simulink model "sys1"  (R2023b)
settings: Solver=VariableStepAuto  StartTime=0.0  StopTime=30e-3  RelTol=1e-3
InitFcn:
  | fs = 100e6;
  | ts = 1 / fs;
values from neighbouring files (symbols this model uses):
  c = 3e8    (= 300000000)    [init_param.m]
  H_az1 = zeros(numSamples,numPulses)    [init_param.m]
  H_az2 = zeros(numSamples,numPulses)    [init_param.m]
  H_ref = fft(conj(fliplr(txChirp)), numSamples)    [init_param.m]
  rawData = rawData + 0.01 * (randn(size(rawData)) + 1j * randn(size(rawData)))    [init_param.m]
  x1 = zeros(size(rawData))    [main.m]
  x2 = zeros(size(x1))    [main.m]
  x3 = zeros(size(x2))    [main.m]
  x4 = zeros(size(x3))    [main.m]
  x5 = zeros(size(x4))    [main.m]
  x6 = zeros(size(x5))    [main.m]
  xx4 = zeros(size(xx3))    [main.m]
  xx5 = zeros(size(xx4))    [main.m]
  xx6 = zeros(size(xx5))    [main.m]
undefined symbols (not defined in the file or in its folder): ffva1156, w2, w3, w4, w5, w6, w7, w8, w9, ww2, ww3, ww4, ww5, ww6, ww7, ww8, ww9, xcku095
libraries: hdlBasic x917, hdlDSPIP x18, dspsrcs4 x12, vmcUtilities x1
(part 9 of 9)

== system sys1/SAR/stream/stream_ifft/stage1/delay/delay1 ==
  in : Inport
  Constant1 : hdlBasic/Constant  const=1  gui_display_data_type=Boolean  arith_type=Boolean  n_bits=16  bin_pt=14  preci_type=Single  exp_width=8  frac_width=24  explicit_period=on  period=ts  XmcBlockStatus=1  maskContainerNames=tabcontainer1  block_type=constant  block_config=sysgen:Constant_config
  Constant3 : hdlBasic/Constant  const=1  gui_display_data_type=Boolean  arith_type=Boolean  n_bits=16  bin_pt=14  preci_type=Single  exp_width=8  frac_width=24  explicit_period=on  period=ts  XmcBlockStatus=1  maskContainerNames=tabcontainer1  block_type=constant  block_config=sysgen:Constant_config
  FIFO : hdlBasic/FIFO  mem_type=Block RAM  performance_options=Standard_FIFO  embedded_registers=off  depth=1K  use_asym_data_widths=off  asym_read_width=32  percent_nbits=1  rst=off  rst_latency=3  en=off  use_dcount=off  use_percent_full_port=off  use_almost_empty=off  almost_empty_thresh=2  use_almost_full=on  use_rd_rst_busy=off  use_wr_rst_busy=off  almost_full_thresh=2^10-3  almost_empty_offset=[]  almost_full_offset=[]  explicit_period=off  period=[]  store_only_valid=[]  init_zero=[]  simulation_type=fast_sim  XmcBlockStatus=1  maskContainerNames=tabcontainer1  block_type=fifo  block_config=sysgen:FIFO_config  block_width=538  block_height=997
      settings: infoedit=[]
  Register2 : hdlBasic/Register  init=0  rst=off  en=on  XmcBlockStatus=1  maskContainerNames=tabcontainer1  block_type=register  block_config=sysgen:Register_config
  out : Outport
  wires:
  FIFO/4 -> Register2/2
  Constant1/1 -> Register2/1
  Register2/1 -> FIFO/3
  Constant3/1 -> FIFO/2
  in/1 -> FIFO/1
  FIFO/1 -> out/1

== system sys1/SAR/stream/stream_ifft/stage2/delay/delay ==
  in : Inport
  Constant1 : hdlBasic/Constant  const=1  gui_display_data_type=Boolean  arith_type=Boolean  n_bits=16  bin_pt=14  preci_type=Single  exp_width=8  frac_width=24  explicit_period=on  period=ts  XmcBlockStatus=1  maskContainerNames=tabcontainer1  block_type=constant  block_config=sysgen:Constant_config
  Constant3 : hdlBasic/Constant  const=1  gui_display_data_type=Boolean  arith_type=Boolean  n_bits=16  bin_pt=14  preci_type=Single  exp_width=8  frac_width=24  explicit_period=on  period=ts  XmcBlockStatus=1  maskContainerNames=tabcontainer1  block_type=constant  block_config=sysgen:Constant_config
  FIFO : hdlBasic/FIFO  mem_type=Block RAM  performance_options=Standard_FIFO  embedded_registers=off  depth=2K  use_asym_data_widths=off  asym_read_width=32  percent_nbits=1  rst=off  rst_latency=3  en=off  use_dcount=off  use_percent_full_port=off  use_almost_empty=off  almost_empty_thresh=2  use_almost_full=on  use_rd_rst_busy=off  use_wr_rst_busy=off  almost_full_thresh=2^11-3  almost_empty_offset=[]  almost_full_offset=[]  explicit_period=off  period=[]  store_only_valid=[]  init_zero=[]  simulation_type=fast_sim  XmcBlockStatus=1  maskContainerNames=tabcontainer1  block_type=fifo  block_config=sysgen:FIFO_config  block_width=538  block_height=997
      settings: infoedit=[]
  Register2 : hdlBasic/Register  init=0  rst=off  en=on  XmcBlockStatus=1  maskContainerNames=tabcontainer1  block_type=register  block_config=sysgen:Register_config
  out : Outport
  wires:
  FIFO/4 -> Register2/2
  Constant1/1 -> Register2/1
  Register2/1 -> FIFO/3
  Constant3/1 -> FIFO/2
  in/1 -> FIFO/1
  FIFO/1 -> out/1

== system sys1/SAR/stream/stream_ifft/stage2/delay/delay1 ==
  in : Inport
  Constant1 : hdlBasic/Constant  const=1  gui_display_data_type=Boolean  arith_type=Boolean  n_bits=16  bin_pt=14  preci_type=Single  exp_width=8  frac_width=24  explicit_period=on  period=ts  XmcBlockStatus=1  maskContainerNames=tabcontainer1  block_type=constant  block_config=sysgen:Constant_config
  Constant3 : hdlBasic/Constant  const=1  gui_display_data_type=Boolean  arith_type=Boolean  n_bits=16  bin_pt=14  preci_type=Single  exp_width=8  frac_width=24  explicit_period=on  period=ts  XmcBlockStatus=1  maskContainerNames=tabcontainer1  block_type=constant  block_config=sysgen:Constant_config
  FIFO : hdlBasic/FIFO  mem_type=Block RAM  performance_options=Standard_FIFO  embedded_registers=off  depth=2K  use_asym_data_widths=off  asym_read_width=32  percent_nbits=1  rst=off  rst_latency=3  en=off  use_dcount=off  use_percent_full_port=off  use_almost_empty=off  almost_empty_thresh=2  use_almost_full=on  use_rd_rst_busy=off  use_wr_rst_busy=off  almost_full_thresh=2^11-3  almost_empty_offset=[]  almost_full_offset=[]  explicit_period=off  period=[]  store_only_valid=[]  init_zero=[]  simulation_type=fast_sim  XmcBlockStatus=1  maskContainerNames=tabcontainer1  block_type=fifo  block_config=sysgen:FIFO_config  block_width=538  block_height=997
      settings: infoedit=[]
  Register2 : hdlBasic/Register  init=0  rst=off  en=on  XmcBlockStatus=1  maskContainerNames=tabcontainer1  block_type=register  block_config=sysgen:Register_config
  out : Outport
  wires:
  FIFO/1 -> out/1
  in/1 -> FIFO/1
  Constant3/1 -> FIFO/2
  Register2/1 -> FIFO/3
  Constant1/1 -> Register2/1
  FIFO/4 -> Register2/2

== system sys1/SAR/stream/stream_ifft/stage3/delay/delay ==
  in : Inport
  Constant1 : hdlBasic/Constant  const=1  gui_display_data_type=Boolean  arith_type=Boolean  n_bits=16  bin_pt=14  preci_type=Single  exp_width=8  frac_width=24  explicit_period=on  period=ts  XmcBlockStatus=1  maskContainerNames=tabcontainer1  block_type=constant  block_config=sysgen:Constant_config
  Constant3 : hdlBasic/Constant  const=1  gui_display_data_type=Boolean  arith_type=Boolean  n_bits=16  bin_pt=14  preci_type=Single  exp_width=8  frac_width=24  explicit_period=on  period=ts  XmcBlockStatus=1  maskContainerNames=tabcontainer1  block_type=constant  block_config=sysgen:Constant_config
  FIFO : hdlBasic/FIFO  mem_type=Block RAM  performance_options=Standard_FIFO  embedded_registers=off  depth=4K  use_asym_data_widths=off  asym_read_width=32  percent_nbits=1  rst=off  rst_latency=3  en=off  use_dcount=off  use_percent_full_port=off  use_almost_empty=off  almost_empty_thresh=2  use_almost_full=on  use_rd_rst_busy=off  use_wr_rst_busy=off  almost_full_thresh=2^12-3  almost_empty_offset=[]  almost_full_offset=[]  explicit_period=off  period=[]  store_only_valid=[]  init_zero=[]  simulation_type=fast_sim  XmcBlockStatus=1  maskContainerNames=tabcontainer1  block_type=fifo  block_config=sysgen:FIFO_config  block_width=538  block_height=997
      settings: infoedit=[]
  Register2 : hdlBasic/Register  init=0  rst=off  en=on  XmcBlockStatus=1  maskContainerNames=tabcontainer1  block_type=register  block_config=sysgen:Register_config
  out : Outport
  wires:
  FIFO/1 -> out/1
  in/1 -> FIFO/1
  Constant3/1 -> FIFO/2
  Register2/1 -> FIFO/3
  Constant1/1 -> Register2/1
  FIFO/4 -> Register2/2

== system sys1/SAR/stream/stream_ifft/stage3/delay/delay1 ==
  in : Inport
  Constant1 : hdlBasic/Constant  const=1  gui_display_data_type=Boolean  arith_type=Boolean  n_bits=16  bin_pt=14  preci_type=Single  exp_width=8  frac_width=24  explicit_period=on  period=ts  XmcBlockStatus=1  maskContainerNames=tabcontainer1  block_type=constant  block_config=sysgen:Constant_config
  Constant3 : hdlBasic/Constant  const=1  gui_display_data_type=Boolean  arith_type=Boolean  n_bits=16  bin_pt=14  preci_type=Single  exp_width=8  frac_width=24  explicit_period=on  period=ts  XmcBlockStatus=1  maskContainerNames=tabcontainer1  block_type=constant  block_config=sysgen:Constant_config
  FIFO : hdlBasic/FIFO  mem_type=Block RAM  performance_options=Standard_FIFO  embedded_registers=off  depth=4K  use_asym_data_widths=off  asym_read_width=32  percent_nbits=1  rst=off  rst_latency=3  en=off  use_dcount=off  use_percent_full_port=off  use_almost_empty=off  almost_empty_thresh=2  use_almost_full=on  use_rd_rst_busy=off  use_wr_rst_busy=off  almost_full_thresh=2^12-3  almost_empty_offset=[]  almost_full_offset=[]  explicit_period=off  period=[]  store_only_valid=[]  init_zero=[]  simulation_type=fast_sim  XmcBlockStatus=1  maskContainerNames=tabcontainer1  block_type=fifo  block_config=sysgen:FIFO_config  block_width=538  block_height=997
      settings: infoedit=[]
  Register2 : hdlBasic/Register  init=0  rst=off  en=on  XmcBlockStatus=1  maskContainerNames=tabcontainer1  block_type=register  block_config=sysgen:Register_config
  out : Outport
  wires:
  FIFO/4 -> Register2/2
  Constant1/1 -> Register2/1
  Register2/1 -> FIFO/3
  Constant3/1 -> FIFO/2
  in/1 -> FIFO/1
  FIFO/1 -> out/1

== system sys1/SAR/stream/stream_ifft/stage4/delay/delay ==
  in : Inport
  Constant1 : hdlBasic/Constant  const=1  gui_display_data_type=Boolean  arith_type=Boolean  n_bits=16  bin_pt=14  preci_type=Single  exp_width=8  frac_width=24  explicit_period=on  period=ts  XmcBlockStatus=1  maskContainerNames=tabcontainer1  block_type=constant  block_config=sysgen:Constant_config
  Constant3 : hdlBasic/Constant  const=1  gui_display_data_type=Boolean  arith_type=Boolean  n_bits=16  bin_pt=14  preci_type=Single  exp_width=8  frac_width=24  explicit_period=on  period=ts  XmcBlockStatus=1  maskContainerNames=tabcontainer1  block_type=constant  block_config=sysgen:Constant_config
  FIFO : hdlBasic/FIFO  mem_type=Block RAM  performance_options=Standard_FIFO  embedded_registers=off  depth=8K  use_asym_data_widths=off  asym_read_width=32  percent_nbits=1  rst=off  rst_latency=3  en=off  use_dcount=off  use_percent_full_port=off  use_almost_empty=off  almost_empty_thresh=2  use_almost_full=on  use_rd_rst_busy=off  use_wr_rst_busy=off  almost_full_thresh=2^13-3  almost_empty_offset=[]  almost_full_offset=[]  explicit_period=off  period=[]  store_only_valid=[]  init_zero=[]  simulation_type=fast_sim  XmcBlockStatus=1  maskContainerNames=tabcontainer1  block_type=fifo  block_config=sysgen:FIFO_config  block_width=538  block_height=997
      settings: infoedit=[]
  Register2 : hdlBasic/Register  init=0  rst=off  en=on  XmcBlockStatus=1  maskContainerNames=tabcontainer1  block_type=register  block_config=sysgen:Register_config
  out : Outport
  wires:
  FIFO/4 -> Register2/2
  Constant1/1 -> Register2/1
  Register2/1 -> FIFO/3
  Constant3/1 -> FIFO/2
  in/1 -> FIFO/1
  FIFO/1 -> out/1

== system sys1/SAR/stream/stream_ifft/stage4/delay/delay1 ==
  in : Inport
  Constant1 : hdlBasic/Constant  const=1  gui_display_data_type=Boolean  arith_type=Boolean  n_bits=16  bin_pt=14  preci_type=Single  exp_width=8  frac_width=24  explicit_period=on  period=ts  XmcBlockStatus=1  maskContainerNames=tabcontainer1  block_type=constant  block_config=sysgen:Constant_config
  Constant3 : hdlBasic/Constant  const=1  gui_display_data_type=Boolean  arith_type=Boolean  n_bits=16  bin_pt=14  preci_type=Single  exp_width=8  frac_width=24  explicit_period=on  period=ts  XmcBlockStatus=1  maskContainerNames=tabcontainer1  block_type=constant  block_config=sysgen:Constant_config
  FIFO : hdlBasic/FIFO  mem_type=Block RAM  performance_options=Standard_FIFO  embedded_registers=off  depth=8K  use_asym_data_widths=off  asym_read_width=32  percent_nbits=1  rst=off  rst_latency=3  en=off  use_dcount=off  use_percent_full_port=off  use_almost_empty=off  almost_empty_thresh=2  use_almost_full=on  use_rd_rst_busy=off  use_wr_rst_busy=off  almost_full_thresh=2^13-3  almost_empty_offset=[]  almost_full_offset=[]  explicit_period=off  period=[]  store_only_valid=[]  init_zero=[]  simulation_type=fast_sim  XmcBlockStatus=1  maskContainerNames=tabcontainer1  block_type=fifo  block_config=sysgen:FIFO_config  block_width=538  block_height=997
      settings: infoedit=[]
  Register2 : hdlBasic/Register  init=0  rst=off  en=on  XmcBlockStatus=1  maskContainerNames=tabcontainer1  block_type=register  block_config=sysgen:Register_config
  out : Outport
  wires:
  FIFO/1 -> out/1
  in/1 -> FIFO/1
  Constant3/1 -> FIFO/2
  Register2/1 -> FIFO/3
  Constant1/1 -> Register2/1
  FIFO/4 -> Register2/2

== system sys1/SAR/stream/stream_ifft/stage5/delay/delay ==
  in : Inport
  Constant1 : hdlBasic/Constant  const=1  gui_display_data_type=Boolean  arith_type=Boolean  n_bits=16  bin_pt=14  preci_type=Single  exp_width=8  frac_width=24  explicit_period=on  period=ts  XmcBlockStatus=1  maskContainerNames=tabcontainer1  block_type=constant  block_config=sysgen:Constant_config
  Constant3 : hdlBasic/Constant  const=1  gui_display_data_type=Boolean  arith_type=Boolean  n_bits=16  bin_pt=14  preci_type=Single  exp_width=8  frac_width=24  explicit_period=on  period=ts  XmcBlockStatus=1  maskContainerNames=tabcontainer1  block_type=constant  block_config=sysgen:Constant_config
  FIFO : hdlBasic/FIFO  mem_type=Block RAM  performance_options=Standard_FIFO  embedded_registers=off  depth=16K  use_asym_data_widths=off  asym_read_width=32  percent_nbits=1  rst=off  rst_latency=3  en=off  use_dcount=off  use_percent_full_port=off  use_almost_empty=off  almost_empty_thresh=2  use_almost_full=on  use_rd_rst_busy=off  use_wr_rst_busy=off  almost_full_thresh=2^14-3  almost_empty_offset=[]  almost_full_offset=[]  explicit_period=off  period=[]  store_only_valid=[]  init_zero=[]  simulation_type=fast_sim  XmcBlockStatus=1  maskContainerNames=tabcontainer1  block_type=fifo  block_config=sysgen:FIFO_config  block_width=538  block_height=997
      settings: infoedit=[]
  Register2 : hdlBasic/Register  init=0  rst=off  en=on  XmcBlockStatus=1  maskContainerNames=tabcontainer1  block_type=register  block_config=sysgen:Register_config
  out : Outport
  wires:
  FIFO/1 -> out/1
  in/1 -> FIFO/1
  Constant3/1 -> FIFO/2
  Register2/1 -> FIFO/3
  Constant1/1 -> Register2/1
  FIFO/4 -> Register2/2

== system sys1/SAR/stream/stream_ifft/stage5/delay/delay1 ==
  in : Inport
  Constant1 : hdlBasic/Constant  const=1  gui_display_data_type=Boolean  arith_type=Boolean  n_bits=16  bin_pt=14  preci_type=Single  exp_width=8  frac_width=24  explicit_period=on  period=ts  XmcBlockStatus=1  maskContainerNames=tabcontainer1  block_type=constant  block_config=sysgen:Constant_config
  Constant3 : hdlBasic/Constant  const=1  gui_display_data_type=Boolean  arith_type=Boolean  n_bits=16  bin_pt=14  preci_type=Single  exp_width=8  frac_width=24  explicit_period=on  period=ts  XmcBlockStatus=1  maskContainerNames=tabcontainer1  block_type=constant  block_config=sysgen:Constant_config
  FIFO : hdlBasic/FIFO  mem_type=Block RAM  performance_options=Standard_FIFO  embedded_registers=off  depth=16K  use_asym_data_widths=off  asym_read_width=32  percent_nbits=1  rst=off  rst_latency=3  en=off  use_dcount=off  use_percent_full_port=off  use_almost_empty=off  almost_empty_thresh=2  use_almost_full=on  use_rd_rst_busy=off  use_wr_rst_busy=off  almost_full_thresh=2^14-3  almost_empty_offset=[]  almost_full_offset=[]  explicit_period=off  period=[]  store_only_valid=[]  init_zero=[]  simulation_type=fast_sim  XmcBlockStatus=1  maskContainerNames=tabcontainer1  block_type=fifo  block_config=sysgen:FIFO_config  block_width=538  block_height=997
      settings: infoedit=[]
  Register2 : hdlBasic/Register  init=0  rst=off  en=on  XmcBlockStatus=1  maskContainerNames=tabcontainer1  block_type=register  block_config=sysgen:Register_config
  out : Outport
  wires:
  FIFO/4 -> Register2/2
  Constant1/1 -> Register2/1
  Register2/1 -> FIFO/3
  Constant3/1 -> FIFO/2
  in/1 -> FIFO/1
  FIFO/1 -> out/1

== system sys1/SAR/stream/stream_ifft/stage6/delay/delay ==
  in : Inport
  Constant1 : hdlBasic/Constant  const=1  gui_display_data_type=Boolean  arith_type=Boolean  n_bits=16  bin_pt=14  preci_type=Single  exp_width=8  frac_width=24  explicit_period=on  period=ts  XmcBlockStatus=1  maskContainerNames=tabcontainer1  block_type=constant  block_config=sysgen:Constant_config
  Constant3 : hdlBasic/Constant  const=1  gui_display_data_type=Boolean  arith_type=Boolean  n_bits=16  bin_pt=14  preci_type=Single  exp_width=8  frac_width=24  explicit_period=on  period=ts  XmcBlockStatus=1  maskContainerNames=tabcontainer1  block_type=constant  block_config=sysgen:Constant_config
  FIFO : hdlBasic/FIFO  mem_type=Block RAM  performance_options=Standard_FIFO  embedded_registers=off  depth=32K  use_asym_data_widths=off  asym_read_width=32  percent_nbits=1  rst=off  rst_latency=3  en=off  use_dcount=off  use_percent_full_port=off  use_almost_empty=off  almost_empty_thresh=2  use_almost_full=on  use_rd_rst_busy=off  use_wr_rst_busy=off  almost_full_thresh=2^15-3  almost_empty_offset=[]  almost_full_offset=[]  explicit_period=off  period=[]  store_only_valid=[]  init_zero=[]  simulation_type=fast_sim  XmcBlockStatus=1  maskContainerNames=tabcontainer1  block_type=fifo  block_config=sysgen:FIFO_config  block_width=538  block_height=997
      settings: infoedit=[]
  Register2 : hdlBasic/Register  init=0  rst=off  en=on  XmcBlockStatus=1  maskContainerNames=tabcontainer1  block_type=register  block_config=sysgen:Register_config
  out : Outport
  wires:
  FIFO/4 -> Register2/2
  Constant1/1 -> Register2/1
  Register2/1 -> FIFO/3
  Constant3/1 -> FIFO/2
  in/1 -> FIFO/1
  FIFO/1 -> out/1

== system sys1/SAR/stream/stream_ifft/stage6/delay/delay1 ==
  in : Inport
  Constant1 : hdlBasic/Constant  const=1  gui_display_data_type=Boolean  arith_type=Boolean  n_bits=16  bin_pt=14  preci_type=Single  exp_width=8  frac_width=24  explicit_period=on  period=ts  XmcBlockStatus=1  maskContainerNames=tabcontainer1  block_type=constant  block_config=sysgen:Constant_config
  Constant3 : hdlBasic/Constant  const=1  gui_display_data_type=Boolean  arith_type=Boolean  n_bits=16  bin_pt=14  preci_type=Single  exp_width=8  frac_width=24  explicit_period=on  period=ts  XmcBlockStatus=1  maskContainerNames=tabcontainer1  block_type=constant  block_config=sysgen:Constant_config
  FIFO : hdlBasic/FIFO  mem_type=Block RAM  performance_options=Standard_FIFO  embedded_registers=off  depth=32K  use_asym_data_widths=off  asym_read_width=32  percent_nbits=1  rst=off  rst_latency=3  en=off  use_dcount=off  use_percent_full_port=off  use_almost_empty=off  almost_empty_thresh=2  use_almost_full=on  use_rd_rst_busy=off  use_wr_rst_busy=off  almost_full_thresh=2^15-3  almost_empty_offset=[]  almost_full_offset=[]  explicit_period=off  period=[]  store_only_valid=[]  init_zero=[]  simulation_type=fast_sim  XmcBlockStatus=1  maskContainerNames=tabcontainer1  block_type=fifo  block_config=sysgen:FIFO_config  block_width=538  block_height=997
      settings: infoedit=[]
  Register2 : hdlBasic/Register  init=0  rst=off  en=on  XmcBlockStatus=1  maskContainerNames=tabcontainer1  block_type=register  block_config=sysgen:Register_config
  out : Outport
  wires:
  FIFO/1 -> out/1
  in/1 -> FIFO/1
  Constant3/1 -> FIFO/2
  Register2/1 -> FIFO/3
  Constant1/1 -> Register2/1
  FIFO/4 -> Register2/2

== system sys1/SAR/stream/stream_ifft/stage7/delay/delay ==
  in : Inport
  Constant1 : hdlBasic/Constant  const=1  gui_display_data_type=Boolean  arith_type=Boolean  n_bits=16  bin_pt=14  preci_type=Single  exp_width=8  frac_width=24  explicit_period=on  period=ts  XmcBlockStatus=1  maskContainerNames=tabcontainer1  block_type=constant  block_config=sysgen:Constant_config
  Constant3 : hdlBasic/Constant  const=1  gui_display_data_type=Boolean  arith_type=Boolean  n_bits=16  bin_pt=14  preci_type=Single  exp_width=8  frac_width=24  explicit_period=on  period=ts  XmcBlockStatus=1  maskContainerNames=tabcontainer1  block_type=constant  block_config=sysgen:Constant_config
  FIFO : hdlBasic/FIFO  mem_type=Block RAM  performance_options=Standard_FIFO  embedded_registers=off  depth=64K  use_asym_data_widths=off  asym_read_width=32  percent_nbits=1  rst=off  rst_latency=3  en=off  use_dcount=off  use_percent_full_port=off  use_almost_empty=off  almost_empty_thresh=2  use_almost_full=on  use_rd_rst_busy=off  use_wr_rst_busy=off  almost_full_thresh=2^16-3  almost_empty_offset=[]  almost_full_offset=[]  explicit_period=off  period=[]  store_only_valid=[]  init_zero=[]  simulation_type=fast_sim  XmcBlockStatus=1  maskContainerNames=tabcontainer1  block_type=fifo  block_config=sysgen:FIFO_config  block_width=538  block_height=997
      settings: infoedit=[]
  Register2 : hdlBasic/Register  init=0  rst=off  en=on  XmcBlockStatus=1  maskContainerNames=tabcontainer1  block_type=register  block_config=sysgen:Register_config
  out : Outport
  wires:
  FIFO/1 -> out/1
  in/1 -> FIFO/1
  Constant3/1 -> FIFO/2
  Register2/1 -> FIFO/3
  Constant1/1 -> Register2/1
  FIFO/4 -> Register2/2

== system sys1/SAR/stream/stream_ifft/stage7/delay/delay1 ==
  in : Inport
  Constant1 : hdlBasic/Constant  const=1  gui_display_data_type=Boolean  arith_type=Boolean  n_bits=16  bin_pt=14  preci_type=Single  exp_width=8  frac_width=24  explicit_period=on  period=ts  XmcBlockStatus=1  maskContainerNames=tabcontainer1  block_type=constant  block_config=sysgen:Constant_config
  Constant3 : hdlBasic/Constant  const=1  gui_display_data_type=Boolean  arith_type=Boolean  n_bits=16  bin_pt=14  preci_type=Single  exp_width=8  frac_width=24  explicit_period=on  period=ts  XmcBlockStatus=1  maskContainerNames=tabcontainer1  block_type=constant  block_config=sysgen:Constant_config
  FIFO : hdlBasic/FIFO  mem_type=Block RAM  performance_options=Standard_FIFO  embedded_registers=off  depth=64K  use_asym_data_widths=off  asym_read_width=32  percent_nbits=1  rst=off  rst_latency=3  en=off  use_dcount=off  use_percent_full_port=off  use_almost_empty=off  almost_empty_thresh=2  use_almost_full=on  use_rd_rst_busy=off  use_wr_rst_busy=off  almost_full_thresh=2^16-3  almost_empty_offset=[]  almost_full_offset=[]  explicit_period=off  period=[]  store_only_valid=[]  init_zero=[]  simulation_type=fast_sim  XmcBlockStatus=1  maskContainerNames=tabcontainer1  block_type=fifo  block_config=sysgen:FIFO_config  block_width=538  block_height=997
      settings: infoedit=[]
  Register2 : hdlBasic/Register  init=0  rst=off  en=on  XmcBlockStatus=1  maskContainerNames=tabcontainer1  block_type=register  block_config=sysgen:Register_config
  out : Outport
  wires:
  FIFO/4 -> Register2/2
  Constant1/1 -> Register2/1
  Register2/1 -> FIFO/3
  Constant3/1 -> FIFO/2
  in/1 -> FIFO/1
  FIFO/1 -> out/1

== system sys1/SAR/stream/stream_ifft/stage8/delay/delay ==
  in : Inport
  Constant1 : hdlBasic/Constant  const=1  gui_display_data_type=Boolean  arith_type=Boolean  n_bits=16  bin_pt=14  preci_type=Single  exp_width=8  frac_width=24  explicit_period=on  period=ts  XmcBlockStatus=1  maskContainerNames=tabcontainer1  block_type=constant  block_config=sysgen:Constant_config
  Constant3 : hdlBasic/Constant  const=1  gui_display_data_type=Boolean  arith_type=Boolean  n_bits=16  bin_pt=14  preci_type=Single  exp_width=8  frac_width=24  explicit_period=on  period=ts  XmcBlockStatus=1  maskContainerNames=tabcontainer1  block_type=constant  block_config=sysgen:Constant_config
  FIFO : hdlBasic/FIFO  mem_type=Block RAM  performance_options=Standard_FIFO  embedded_registers=off  depth=128K  use_asym_data_widths=off  asym_read_width=32  percent_nbits=1  rst=off  rst_latency=3  en=off  use_dcount=off  use_percent_full_port=off  use_almost_empty=off  almost_empty_thresh=2  use_almost_full=on  use_rd_rst_busy=off  use_wr_rst_busy=off  almost_full_thresh=2^17-3  almost_empty_offset=[]  almost_full_offset=[]  explicit_period=off  period=[]  store_only_valid=[]  init_zero=[]  simulation_type=fast_sim  XmcBlockStatus=1  maskContainerNames=tabcontainer1  block_type=fifo  block_config=sysgen:FIFO_config  block_width=538  block_height=997
      settings: infoedit=[]
  Register2 : hdlBasic/Register  init=0  rst=off  en=on  XmcBlockStatus=1  maskContainerNames=tabcontainer1  block_type=register  block_config=sysgen:Register_config
  out : Outport
  wires:
  FIFO/4 -> Register2/2
  Constant1/1 -> Register2/1
  Register2/1 -> FIFO/3
  Constant3/1 -> FIFO/2
  in/1 -> FIFO/1
  FIFO/1 -> out/1

== system sys1/SAR/stream/stream_ifft/stage8/delay/delay1 ==
  in : Inport
  Constant1 : hdlBasic/Constant  const=1  gui_display_data_type=Boolean  arith_type=Boolean  n_bits=16  bin_pt=14  preci_type=Single  exp_width=8  frac_width=24  explicit_period=on  period=ts  XmcBlockStatus=1  maskContainerNames=tabcontainer1  block_type=constant  block_config=sysgen:Constant_config
  Constant3 : hdlBasic/Constant  const=1  gui_display_data_type=Boolean  arith_type=Boolean  n_bits=16  bin_pt=14  preci_type=Single  exp_width=8  frac_width=24  explicit_period=on  period=ts  XmcBlockStatus=1  maskContainerNames=tabcontainer1  block_type=constant  block_config=sysgen:Constant_config
  FIFO : hdlBasic/FIFO  mem_type=Block RAM  performance_options=Standard_FIFO  embedded_registers=off  depth=128K  use_asym_data_widths=off  asym_read_width=32  percent_nbits=1  rst=off  rst_latency=3  en=off  use_dcount=off  use_percent_full_port=off  use_almost_empty=off  almost_empty_thresh=2  use_almost_full=on  use_rd_rst_busy=off  use_wr_rst_busy=off  almost_full_thresh=2^17-3  almost_empty_offset=[]  almost_full_offset=[]  explicit_period=off  period=[]  store_only_valid=[]  init_zero=[]  simulation_type=fast_sim  XmcBlockStatus=1  maskContainerNames=tabcontainer1  block_type=fifo  block_config=sysgen:FIFO_config  block_width=538  block_height=997
      settings: infoedit=[]
  Register2 : hdlBasic/Register  init=0  rst=off  en=on  XmcBlockStatus=1  maskContainerNames=tabcontainer1  block_type=register  block_config=sysgen:Register_config
  out : Outport
  wires:
  FIFO/1 -> out/1
  in/1 -> FIFO/1
  Constant3/1 -> FIFO/2
  Register2/1 -> FIFO/3
  Constant1/1 -> Register2/1
  FIFO/4 -> Register2/2

== system sys1/SAR/stream/stream_ifft/stage9/delay/delay ==
  in : Inport
  Constant1 : hdlBasic/Constant  const=1  gui_display_data_type=Boolean  arith_type=Boolean  n_bits=16  bin_pt=14  preci_type=Single  exp_width=8  frac_width=24  explicit_period=on  period=ts  XmcBlockStatus=1  maskContainerNames=tabcontainer1  block_type=constant  block_config=sysgen:Constant_config
  Constant3 : hdlBasic/Constant  const=1  gui_display_data_type=Boolean  arith_type=Boolean  n_bits=16  bin_pt=14  preci_type=Single  exp_width=8  frac_width=24  explicit_period=on  period=ts  XmcBlockStatus=1  maskContainerNames=tabcontainer1  block_type=constant  block_config=sysgen:Constant_config
  FIFO : hdlBasic/FIFO  mem_type=Block RAM  performance_options=Standard_FIFO  embedded_registers=off  depth=128K  use_asym_data_widths=off  asym_read_width=32  percent_nbits=1  rst=off  rst_latency=3  en=off  use_dcount=off  use_percent_full_port=off  use_almost_empty=off  almost_empty_thresh=2  use_almost_full=on  use_rd_rst_busy=off  use_wr_rst_busy=off  almost_full_thresh=2^17-3  almost_empty_offset=[]  almost_full_offset=[]  explicit_period=off  period=[]  store_only_valid=[]  init_zero=[]  simulation_type=fast_sim  XmcBlockStatus=1  maskContainerNames=tabcontainer1  block_type=fifo  block_config=sysgen:FIFO_config  block_width=538  block_height=997
      settings: infoedit=[]
  Register2 : hdlBasic/Register  init=0  rst=off  en=on  XmcBlockStatus=1  maskContainerNames=tabcontainer1  block_type=register  block_config=sysgen:Register_config
  out : Outport
  wires:
  FIFO/1 -> out/1
  in/1 -> FIFO/1
  Constant3/1 -> FIFO/2
  Register2/1 -> FIFO/3
  Constant1/1 -> Register2/1
  FIFO/4 -> Register2/2

== system sys1/SAR/stream/stream_ifft/stage9/delay/delay1 ==
  in : Inport
  Constant1 : hdlBasic/Constant  const=1  gui_display_data_type=Boolean  arith_type=Boolean  n_bits=16  bin_pt=14  preci_type=Single  exp_width=8  frac_width=24  explicit_period=on  period=ts  XmcBlockStatus=1  maskContainerNames=tabcontainer1  block_type=constant  block_config=sysgen:Constant_config
  Constant3 : hdlBasic/Constant  const=1  gui_display_data_type=Boolean  arith_type=Boolean  n_bits=16  bin_pt=14  preci_type=Single  exp_width=8  frac_width=24  explicit_period=on  period=ts  XmcBlockStatus=1  maskContainerNames=tabcontainer1  block_type=constant  block_config=sysgen:Constant_config
  FIFO : hdlBasic/FIFO  mem_type=Block RAM  performance_options=Standard_FIFO  embedded_registers=off  depth=128K  use_asym_data_widths=off  asym_read_width=32  percent_nbits=1  rst=off  rst_latency=3  en=off  use_dcount=off  use_percent_full_port=off  use_almost_empty=off  almost_empty_thresh=2  use_almost_full=on  use_rd_rst_busy=off  use_wr_rst_busy=off  almost_full_thresh=2^17-3  almost_empty_offset=[]  almost_full_offset=[]  explicit_period=off  period=[]  store_only_valid=[]  init_zero=[]  simulation_type=fast_sim  XmcBlockStatus=1  maskContainerNames=tabcontainer1  block_type=fifo  block_config=sysgen:FIFO_config  block_width=538  block_height=997
      settings: infoedit=[]
  Register2 : hdlBasic/Register  init=0  rst=off  en=on  XmcBlockStatus=1  maskContainerNames=tabcontainer1  block_type=register  block_config=sysgen:Register_config
  out : Outport
  wires:
  FIFO/4 -> Register2/2
  Constant1/1 -> Register2/1
  Register2/1 -> FIFO/3
  Constant3/1 -> FIFO/2
  in/1 -> FIFO/1
  FIFO/1 -> out/1

== system sys1/SAR/stream/stream_ifft/stage9/delay/delay2 ==
  in : Inport
  Constant1 : hdlBasic/Constant  const=1  gui_display_data_type=Boolean  arith_type=Boolean  n_bits=16  bin_pt=14  preci_type=Single  exp_width=8  frac_width=24  explicit_period=on  period=ts  XmcBlockStatus=1  maskContainerNames=tabcontainer1  block_type=constant  block_config=sysgen:Constant_config
  Constant3 : hdlBasic/Constant  const=1  gui_display_data_type=Boolean  arith_type=Boolean  n_bits=16  bin_pt=14  preci_type=Single  exp_width=8  frac_width=24  explicit_period=on  period=ts  XmcBlockStatus=1  maskContainerNames=tabcontainer1  block_type=constant  block_config=sysgen:Constant_config
  FIFO : hdlBasic/FIFO  mem_type=Block RAM  performance_options=Standard_FIFO  embedded_registers=off  depth=128K  use_asym_data_widths=off  asym_read_width=32  percent_nbits=1  rst=off  rst_latency=3  en=off  use_dcount=off  use_percent_full_port=off  use_almost_empty=off  almost_empty_thresh=2  use_almost_full=on  use_rd_rst_busy=off  use_wr_rst_busy=off  almost_full_thresh=2^17-3  almost_empty_offset=[]  almost_full_offset=[]  explicit_period=off  period=[]  store_only_valid=[]  init_zero=[]  simulation_type=fast_sim  XmcBlockStatus=1  maskContainerNames=tabcontainer1  block_type=fifo  block_config=sysgen:FIFO_config  block_width=538  block_height=997
      settings: infoedit=[]
  Register2 : hdlBasic/Register  init=0  rst=off  en=on  XmcBlockStatus=1  maskContainerNames=tabcontainer1  block_type=register  block_config=sysgen:Register_config
  out : Outport
  wires:
  FIFO/4 -> Register2/2
  Constant1/1 -> Register2/1
  Register2/1 -> FIFO/3
  Constant3/1 -> FIFO/2
  in/1 -> FIFO/1
  FIFO/1 -> out/1

== system sys1/SAR/stream/stream_ifft/stage9/delay/delay3 ==
  in : Inport
  Constant1 : hdlBasic/Constant  const=1  gui_display_data_type=Boolean  arith_type=Boolean  n_bits=16  bin_pt=14  preci_type=Single  exp_width=8  frac_width=24  explicit_period=on  period=ts  XmcBlockStatus=1  maskContainerNames=tabcontainer1  block_type=constant  block_config=sysgen:Constant_config
  Constant3 : hdlBasic/Constant  const=1  gui_display_data_type=Boolean  arith_type=Boolean  n_bits=16  bin_pt=14  preci_type=Single  exp_width=8  frac_width=24  explicit_period=on  period=ts  XmcBlockStatus=1  maskContainerNames=tabcontainer1  block_type=constant  block_config=sysgen:Constant_config
  FIFO : hdlBasic/FIFO  mem_type=Block RAM  performance_options=Standard_FIFO  embedded_registers=off  depth=128K  use_asym_data_widths=off  asym_read_width=32  percent_nbits=1  rst=off  rst_latency=3  en=off  use_dcount=off  use_percent_full_port=off  use_almost_empty=off  almost_empty_thresh=2  use_almost_full=on  use_rd_rst_busy=off  use_wr_rst_busy=off  almost_full_thresh=2^17-3  almost_empty_offset=[]  almost_full_offset=[]  explicit_period=off  period=[]  store_only_valid=[]  init_zero=[]  simulation_type=fast_sim  XmcBlockStatus=1  maskContainerNames=tabcontainer1  block_type=fifo  block_config=sysgen:FIFO_config  block_width=538  block_height=997
      settings: infoedit=[]
  Register2 : hdlBasic/Register  init=0  rst=off  en=on  XmcBlockStatus=1  maskContainerNames=tabcontainer1  block_type=register  block_config=sysgen:Register_config
  out : Outport
  wires:
  FIFO/1 -> out/1
  in/1 -> FIFO/1
  Constant3/1 -> FIFO/2
  Register2/1 -> FIFO/3
  Constant1/1 -> Register2/1
  FIFO/4 -> Register2/2
